simulink model "IN"  (R2017a)
settings: Solver=VariableStepAuto  StartTime=0.0  StopTime=0.1  MaxStep=1e-4  RelTol=1e-3
libraries: powerlib x10
settings Model: Creator=Ahmed  LastModifiedBy=Ahmed

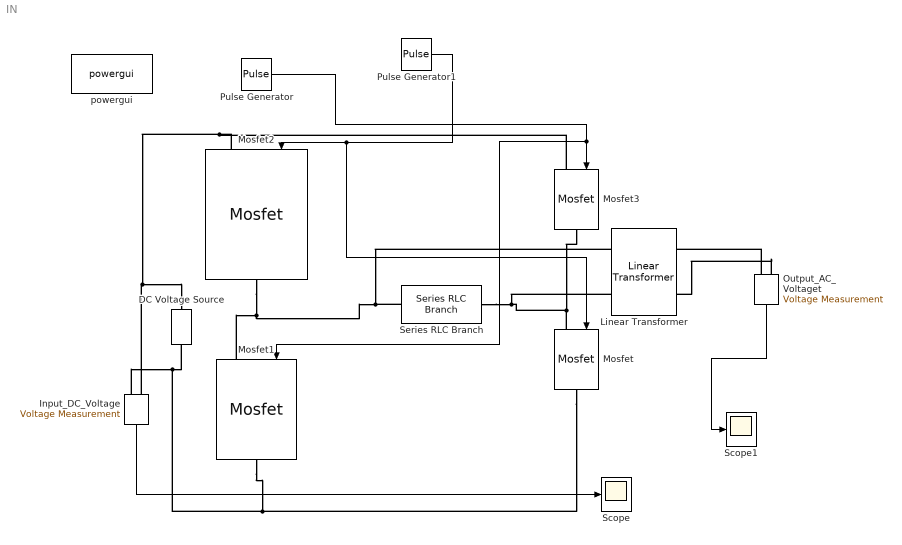
== system IN ==
  DC Voltage Source : powerlib/Electrical Sources/DC Voltage Source  Amplitude=12  Measurements=None
  Input_DC_Voltage : powerlib/Measurements/Voltage Measurement  PhasorSimulation=off  OutputType=Complex  PSBequivalent=0
  Linear Transformer : powerlib/Elements/Linear Transformer  UNITS=SI  NominalPower=[75e3,60]  winding1=[12 0 0]  winding2=[220 0 0]  ThreeWindings=off  winding3=[3.15e+05 315.06 0.088675]  RmLm=[Inf Inf]  Measurements=Winding voltages  DataType=on
  Mosfet{,1..3} (4 alike) : powerlib/Power Electronics/Mosfet  Ron=0.1  Lon=0  Rd=0.01  Vfd=0  IC=0  Rs=1e5  Cs=inf  Measurements=off
  Output_AC_Voltaget : powerlib/Measurements/Voltage Measurement  PhasorSimulation=off  OutputType=Complex  PSBequivalent=0
  Pulse Generator : DiscretePulseGenerator  PulseType=Time based  Amplitude=5  Period=0.02  PulseWidth=50  PhaseDelay=0.01  VectorParams1D=off
  Pulse Generator1 : DiscretePulseGenerator  PulseType=Time based  Amplitude=5  Period=0.02  PulseWidth=50  VectorParams1D=off
  Scope : Scope
  Scope1 : Scope
  Series RLC Branch : powerlib/Elements/Series RLC Branch  LConnTagsString=__new0  RConnTagsString=__new0  BranchType=R  Resistance=5  Inductance=1e-3  SetiL0=off  InitialCurrent=0  Capacitance=1e-6  Setx0=off  InitialVoltage=0  Measurements=None
  powergui : powerlib/powergui  Priority=1  SimulationMode=Continuous  SampleTime=50e-6  frequency=60  Iterations=50  frequencyindice=0  Pbase=100e6  ErrMax=1e-4  UnitsV=kV  UnitsW=MW  buscounter=0  FunctionMessages=off  echomessages=off  EnableUseOfTLC=off  CurrentSourceSwitches=off  DisableSnubberDevices=off  DisableRonSwitches=off  DisableVfSwitches=off  DisplayEquations=off  SolverType=Tustin/Backward Euler (TBE)  Interpol=off  ExternalGateDelay=off  methode=off  Ts=100  x0status=blocks  SPID=on  SwTol=0  HookPort=off  RestoreLinks=warning  ResistiveCurrentMeasurement=off  Frange=[0:2:500]  Ylog=off  Xlog=on  ShowGrid=off  save=off  variable=ZData  structure=0  ZoomFFT=off  StartTime=0.0  cycles=1  DisplayStyle=1  fundamental=60  FreqAxis=off  MaxFrequency=1000  frequencyindicesteady=1  RmsSteady=1  display=off
  wires:
  Pulse Generator1/1 -> Mosfet/1, Mosfet2/1
  Pulse Generator/1 -> Mosfet1/1, Mosfet3/1
  Input_DC_Voltage/1 -> Scope/1
  Output_AC_Voltaget/1 -> Scope1/1
  connections:
  Series RLC Branch/LConn1 -- Mosfet1/LConn1 -- Mosfet2/RConn1 -- Linear Transformer/LConn1
  Series RLC Branch/RConn1 -- Mosfet/LConn1 -- Mosfet3/RConn1 -- Linear Transformer/LConn2
  Input_DC_Voltage/LConn2 -- Mosfet1/RConn1 -- Mosfet/RConn1 -- DC Voltage Source/LConn1
  Input_DC_Voltage/LConn1 -- Mosfet3/LConn1 -- Mosfet2/LConn1 -- DC Voltage Source/RConn1
  Output_AC_Voltaget/LConn2 -- Linear Transformer/RConn1
  Output_AC_Voltaget/LConn1 -- Linear Transformer/RConn2
